simulink model "EemfObserverTest"  (R2026b)
settings: Solver=FixedStepDiscrete  StopTime=emfTestCfg.Duration  FixedStep=emfCfg.Ts
PostLoadFcn:
  | addpath(fullfile(fileparts(get_param(bdroot,'FileName')),'..','build_process'));initialize_emf_test(bdroot);
model workspace (MAT data in the model file):
  emfCfg.Ts = 5e-05
  emfCfg.Rs = 0.5
  emfCfg.Ld = 0.001
  emfCfg.Lq = 0.0012
  emfCfg.Flux = 0.035
  emfCfg.PolePairs = 4
  emfCfg.BandwidthHz = 300
  emfCfg.MinEmf = 1
  emfCfg.MinOmega = 30
  emfCfg.MaxResidual = 1.5
  emfTestCfg.Duration = 0.4
  emfTestCfg.ElectricalSpeed = 200
  emfTestCfg.InitialAngle = 0.4
  emfTestCfg.Id = -2
  emfTestCfg.Iq = 2
  emfTestCfg.Enable = 1
  emfTestCfg.Reset = 0
  emfTestCfg.Direction = []
  pllCfg.Ts = 5e-05
  pllCfg.NaturalFrequency = 40
  pllCfg.Damping = 0.707
  pllCfg.Kp = 355.376960974
  pllCfg.Ki = 63165.468167
  pllCfg.Kaw = 502.654824574
  pllCfg.OmegaMax = 1500
  pllCfg.MinMagnitude = 1
  pllCfg.LockError = 0.12
  pllCfg.LockSamples = 100
  pllCfg.Theta0 = 0
  pllCfg.Omega0 = 0
  testStim.time = []
  testStim.signals.values = [-4.32274967267 -4.38676971045 -4.45035107491 -4.51348740798 -4.57617239607 -4.63839977073 -4.70016330928 -4.76145683541 -4.82227421983 -4.88260938084 -4.94245628499 -5.00180894763 ... (72009 elements, 8001x9)]
  testStim.signals.dimensions = 9
libraries: EmfObserver x1
settings Model: Creator=24322  LastModifiedBy=24322

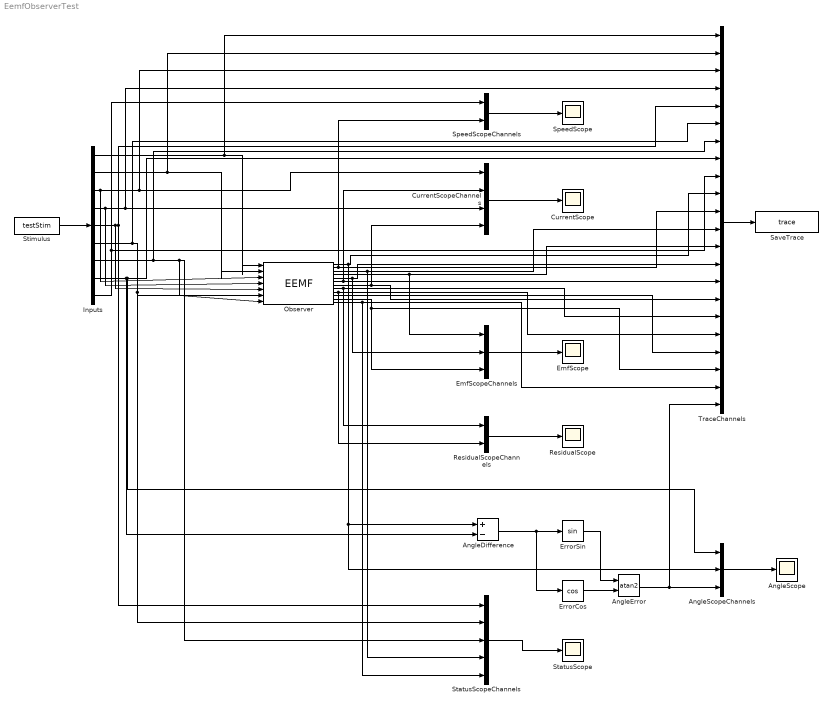
== system EemfObserverTest ==
  AngleDifference : Sum  Inputs=+-
  AngleError : Trigonometry  Operator=atan2
  AngleScope : Scope
  AngleScopeChannels : Mux  Inputs=3
  CurrentScope : Scope
  CurrentScopeChannels : Mux
  EmfScope : Scope
  EmfScopeChannels : Mux  Inputs=3
  ErrorCos : Trigonometry  Operator=cos
  ErrorSin : Trigonometry
  Inputs : Demux  Outputs=9
  Observer : EmfObserver/EEMF  cfg=emfCfg  trackerCfg=pllCfg
  ResidualScope : Scope
  ResidualScopeChannels : Mux  Inputs=2
  SaveTrace : ToWorkspace  VariableName=trace  SaveFormat=Structure With Time  SampleTime=-1
  SpeedScope : Scope
  SpeedScopeChannels : Mux  Inputs=2
  StatusScope : Scope
  StatusScopeChannels : Mux  Inputs=5
  Stimulus : FromWorkspace  VariableName=testStim  SampleTime=emfCfg.Ts  Interpolate=off  OutputAfterFinalValue=Holding final value
  TraceChannels : Mux  Inputs=22
  wires:
  StatusScopeChannels/1 -> StatusScope/1
  ResidualScopeChannels/1 -> ResidualScope/1
  CurrentScopeChannels/1 -> CurrentScope/1
  EmfScopeChannels/1 -> EmfScope/1
  SpeedScopeChannels/1 -> SpeedScope/1
  AngleScopeChannels/1 -> AngleScope/1
  Observer/12 -> TraceChannels/21, StatusScopeChannels/5
  Observer/11 -> TraceChannels/20, EmfScopeChannels/3
  Observer/10 -> TraceChannels/19
  Observer/9 -> TraceChannels/18, ResidualScopeChannels/2
  Observer/8 -> TraceChannels/17, ResidualScopeChannels/1
  Observer/7 -> TraceChannels/16, CurrentScopeChannels/4
  Observer/6 -> TraceChannels/15, CurrentScopeChannels/2
  Observer/5 -> TraceChannels/14, EmfScopeChannels/2
  Observer/4 -> TraceChannels/13, EmfScopeChannels/1
  Observer/3 -> TraceChannels/12, StatusScopeChannels/4
  Observer/2 -> TraceChannels/11, SpeedScopeChannels/2
  Inputs/9 -> TraceChannels/9, SpeedScopeChannels/1
  Inputs/7 -> Observer/7, StatusScopeChannels/3, TraceChannels/7
  Inputs/6 -> Observer/6, StatusScopeChannels/2, TraceChannels/6
  Inputs/5 -> TraceChannels/5, StatusScopeChannels/1, Observer/5
  Inputs/4 -> CurrentScopeChannels/3, TraceChannels/4, Observer/4
  Inputs/3 -> CurrentScopeChannels/1, TraceChannels/3, Observer/3
  Inputs/2 -> Observer/2, TraceChannels/2
  Inputs/1 -> Observer/1, TraceChannels/1
  TraceChannels/1 -> SaveTrace/1
  AngleError/1 -> TraceChannels/22, AngleScopeChannels/3
  ErrorCos/1 -> AngleError/2
  ErrorSin/1 -> AngleError/1
  AngleDifference/1 -> ErrorSin/1, ErrorCos/1
  Inputs/8 -> TraceChannels/8, AngleScopeChannels/1, AngleDifference/2
  Observer/1 -> AngleDifference/1, AngleScopeChannels/2, TraceChannels/10
  Stimulus/1 -> Inputs/1
